simulink model "acf_force_control_adc_trial"  (R2026b)
settings: Solver=ode4  StopTime=0.25  FixedStep=3.3333333333333333e-06
InitFcn:
  | acf_select_actuator(bdroot);
model workspace (MAT data in the model file):
  acfControlVersion = 'force-observer-v1'
  acfImplementation = 'simple'
  acfLayoutVersion = 1
  p : object (value not decoded)
  pCompliant : object (value not decoded)
  pNearContact : object (value not decoded)
  pNoSprings : object (value not decoded)
  pRecommended : object (value not decoded)
symbols that are objects in the model workspace (value not decoded): p
undefined symbols (not defined in the file): DiscIntNeverNeededParam
libraries: sl_discontinuities x1
(part 4 of 4)

== system acf_force_control_adc_trial/Force controller/Coil PI and PID/Normal force PI and PID ==
  error_N : Inport
  anti_windup : Inport  Port=2
  Error to normal deviation : Gain  Gain=-1
  Normal error and anti windup : Sum
  Normal error derivative memory : UnitDelay  SampleTime=p.force.sampleTime
  Normal error filtered derivative : Sum
  Normal error new derivative weight : Gain  Gain=(1-exp(-p.force.sampleTime/p.inertial.derivativeFilter))/p.force.sampleTime
  Normal error old derivative weight : Gain  Gain=exp(-p.force.sampleTime/p.inertial.derivativeFilter)
  Normal error previous sample : UnitDelay  SampleTime=p.force.sampleTime
  Normal error sample increment : Sum  Inputs=+-
  Normal force derivative current : Gain  Gain=-p.inertial.forceKd*double(strcmp(p.coil.strategy,'pid'))
  Normal force error integral : DiscreteIntegrator  SampleTime=p.force.sampleTime  ICPrevOutput=DiscIntNeverNeededParam  ICPrevScaledInput=DiscIntNeverNeededParam
  Normal force integral current : Gain  Gain=-p.inertial.forceKi
  Normal force proportional current : Gain  Gain=-p.inertial.forceKp
  Optional feedback rolloff : DiscreteTransferFcn  Numerator=p.d.feedbackFilter.numerator  Denominator=p.d.feedbackFilter.denominator  InitialStates=p.d.feedbackFilter.initialStates  SampleTime=p.force.sampleTime
  PI and PID correction : Sum  Inputs=+++
  feedback_current_A : Outport
  wires:
  Normal error derivative memory/1 -> Normal error old derivative weight/1
  Normal force proportional current/1 -> PI and PID correction/1
  anti_windup/1 -> Normal error and anti windup/2
  Normal force integral current/1 -> PI and PID correction/2
  Normal error old derivative weight/1 -> Normal error filtered derivative/2
  Error to normal deviation/1 -> Normal error previous sample/1, Normal error and anti windup/1, Normal force proportional current/1, Normal error sample increment/1
  error_N/1 -> Error to normal deviation/1
  Normal error and anti windup/1 -> Normal force error integral/1
  Normal error previous sample/1 -> Normal error sample increment/2
  Normal force error integral/1 -> Normal force integral current/1
  Normal force derivative current/1 -> PI and PID correction/3
  Normal error sample increment/1 -> Normal error new derivative weight/1
  Normal error filtered derivative/1 -> Normal force derivative current/1, Normal error derivative memory/1
  Normal error new derivative weight/1 -> Normal error filtered derivative/1
  PI and PID correction/1 -> Optional feedback rolloff/1
  Optional feedback rolloff/1 -> feedback_current_A/1

== system acf_force_control_adc_trial/Recenter travel/Force settling gate/Fast force variation and dwell ==
  normal_error_N : Inport
  held_slow_stability : Inport  Port=2
  All force stability conditions : Logic  AllPortsSameDT=off  OutDataTypeStr=boolean
  Allowed force variance : Constant  Value=p.robot.forceGate.variation.rmsLimit_N^2
  Cap fast stable count : Saturate  UpperLimit=p.d.variationGate.dwellSamples  LowerLimit=0
  Fast continuous dwell completed : RelationalOperator  OutDataTypeStr=boolean  RndMeth=Simplest  InputSameDT=off
  Fast error sample : ZeroOrderHold  SampleTime=p.force.sampleTime
  Fast force variance : DiscreteTransferFcn  Numerator=p.d.variationGate.varianceNumerator  Denominator=p.d.variationGate.varianceDenominator  SampleTime=p.force.sampleTime
  Fast normal force mean : DiscreteTransferFcn  Numerator=p.d.variationGate.meanNumerator  Denominator=p.d.variationGate.meanDenominator  SampleTime=p.force.sampleTime
  Held slow stability at fast rate : ZeroOrderHold  SampleTime=p.force.sampleTime
  Normal force above target : Gain  Gain=-1
  Normal force deviation : Sum  Inputs=+-
  One more fast stable sample : Bias  Bias=1  SaturateOnIntegerOverflow=off
  Previous fast stable count : UnitDelay  SampleTime=p.force.sampleTime
  RMS force variation : Math  Operator=sqrt
  Required fast dwell count : Constant  Value=p.d.variationGate.dwellSamples
  Reset dwell at every fast instability : Switch  Threshold=.5  SaturateOnIntegerOverflow=off  InputSameDT=off
  Reset fast dwell : Constant  Value=0
  Squared normal force deviation : Math  Operator=square
  Variation acceptable : RelationalOperator  Operator=<=  OutDataTypeStr=boolean  RndMeth=Simplest  InputSameDT=off
  ready_fast : Outport
  mean_error_N : Outport  Port=2
  variation_rms_N : Outport  Port=3
  stable_sample_count : Outport  Port=4
  stable_fast : Outport  Port=5
  wires:
  normal_error_N/1 -> Fast error sample/1
  Fast error sample/1 -> Normal force above target/1
  Normal force above target/1 -> Fast normal force mean/1, Normal force deviation/1
  Fast normal force mean/1 -> Normal force deviation/2, mean_error_N/1
  Normal force deviation/1 -> Squared normal force deviation/1
  Squared normal force deviation/1 -> Fast force variance/1
  Fast force variance/1 -> RMS force variation/1, Variation acceptable/1
  Allowed force variance/1 -> Variation acceptable/2
  held_slow_stability/1 -> Held slow stability at fast rate/1
  Held slow stability at fast rate/1 -> All force stability conditions/1
  Variation acceptable/1 -> All force stability conditions/2
  Previous fast stable count/1 -> One more fast stable sample/1
  One more fast stable sample/1 -> Reset dwell at every fast instability/1
  All force stability conditions/1 -> Reset dwell at every fast instability/2, stable_fast/1
  Reset fast dwell/1 -> Reset dwell at every fast instability/3
  Reset dwell at every fast instability/1 -> Cap fast stable count/1
  Cap fast stable count/1 -> Previous fast stable count/1, Fast continuous dwell completed/1, stable_sample_count/1
  Required fast dwell count/1 -> Fast continuous dwell completed/2
  Fast continuous dwell completed/1 -> ready_fast/1
  RMS force variation/1 -> variation_rms_N/1
